simulink model "MotorCC_V3_R2024b"  (R2024b)
settings: Solver=VariableStepAuto  StartTime=0.0  StopTime=inf  RelTol=1e-3
undefined symbols (not defined in the file or in its folder): LF
libraries: instrumentseriallib x3
settings Model: PacingRate=0.010000  Creator=ignacioalvarado  LastModifiedBy=ignacio
settings OptimizationCC: ReuseModelBlockBuffer=off
settings RTWCC: GPUComputeCapability=3.5
settings ConfigComp: CovBoundaryAbsTol=1.0e-5

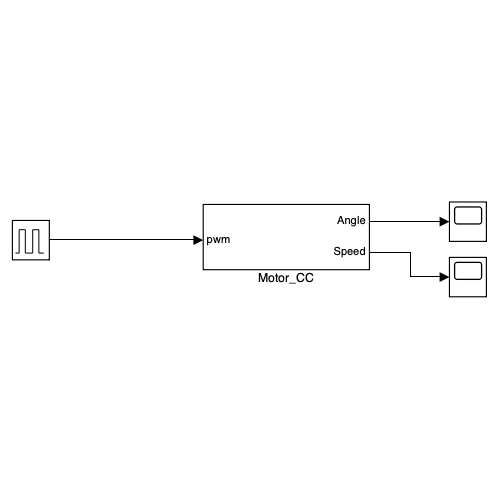
[thumbnail: Simulink's stored preview of the top-level diagram]
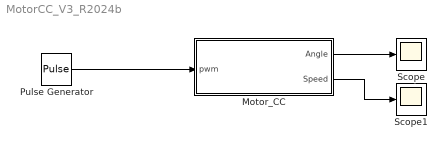
== system MotorCC_V3_R2024b ==
  Motor_CC : Subsystem  InitFcn=|  mask{PortName=Select a serial port}
      | if ismember(get_param(gcb, 'PortName'), {'Select a serial port', 'No serial ports available'})
      |     error('MotorCC:NoSerialPort', 'Connect the Arduino and select its serial port in Motor_CC before running.');
      | end
      mask prompts: PortName "Arduino Port:"
      mask init:
      | % Pass the chosen port to all three Instrument Control Toolbox blocks.
      | block = gcb;
      | selected = get_param(block, 'PortName');
      | if ~ismember(selected, {'Select a serial port', 'No serial ports available'})
      |     set_param([block '/Serial Configuration'], 'Port', selected);
      |     set_param([block '/Serial Send'], 'Port', selected);
      |     set_param([block '/Serial Receive'], 'Port', selected);
      | end
      settings: OpenFcn=|
      | % Refresh the list before showing the mask.
      | block = gcb;
      | if strcmp(get_param(bdroot(block), 'SimulationStatus'), 'stopped')
      |     ports = serialportlist('available');
      |     if isempty(ports)
      |         options = {'No serial ports available'};
      |     else
      |         options = [{'Select a serial port'}, cellstr(ports(:).')];
      |     end
      |     mask = Simulink.Mask.get(block);
      |     port = mask.getParameter('PortName');
      |     selected = get_param(block, 'PortName');
      |     port.TypeOptions = options;
      |     if ~ismember(selected, options)
      |         set_param(block, 'PortName', options{1});
      |     end
      | end
      | open_system(block, 'mask');
      mask TypeOptions PortName: Select a serial port | /dev/tty.Bluetooth-Incoming-Port | /dev/cu.Bluetooth-Incoming-Port | /dev/tty.usbmodem141011 | /dev/cu.usbmodem141011
  Pulse Generator : DiscretePulseGenerator  PulseType=Time based  Amplitude=50  Period=10  PulseWidth=50
  Scope : Scope
  Scope1 : Scope
  wires:
  Pulse Generator/1 -> Motor_CC/1(pwm)
  Motor_CC/1(Angle) -> Scope/1
  Motor_CC/2(Speed) -> Scope1/1

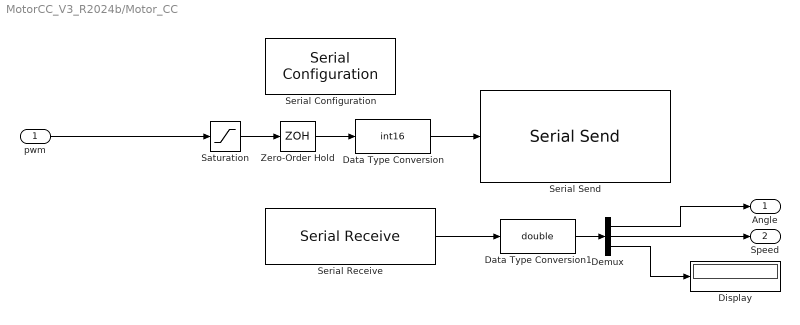
== system MotorCC_V3_R2024b/Motor_CC ==
  pwm : Inport
  Data Type Conversion : DataTypeConversion  OutDataTypeStr=int16  SaturateOnIntegerOverflow=off  RndMeth=Floor  LockScale=on
  Data Type Conversion1 : DataTypeConversion  OutDataTypeStr=double  SaturateOnIntegerOverflow=off  RndMeth=Floor
  Demux : Demux  Outputs=3
  Display : Display
  Saturation : Saturate  UpperLimit=255  LowerLimit=-255
  Serial Configuration : instrumentseriallib/Serial Configuration  Priority=-200000  PortSel=/dev/cu.usbmodem23101  Port=/dev/cu.usbmodem23101  ComPort=/dev/cu.usbmodem23101  BaudRate=115200  DataBits=8  Parity=none  StopBits=1  ByteOrder=little-endian  FlowControl=none  Timeout=10  SimulateUsing=Interpreted execution  BlockInModel=on  aMode=1
  Serial Receive : instrumentseriallib/Serial Receive  Priority=1  PortSel=/dev/cu.usbmodem23101  Port=/dev/cu.usbmodem23101  ComPort=/dev/cu.usbmodem23101  DataType=single  SaveDataType=uint8  ToggleHeader=on  Header='V'  ToggleDataSize=on  DataSize=[1 3]  ToggleTerminator=on  Terminator=LF ('\n')  CustomTerminator=[]  InputFormat=Row major  EnableBlockingMode=on  ActionDataUnavailable=Output last received value  ActionWhenDataUnavailable=Output last received value  CustomValue=0  SampleTime=0.01  SimulateUsing=Interpreted execution  BlockInModel=on  aMode=1
  Serial Send : instrumentseriallib/Serial Send  Priority=1  PortSel=/dev/cu.usbmodem23101  Port=/dev/cu.usbmodem23101  ComPort=/dev/cu.usbmodem23101  Header='A'  Terminator=LF ('\n')  CustomTerminator=[]  EnableBlockingMode=on  SimulateUsing=Interpreted execution  BlockInModel=on  aMode=1
  Zero-Order Hold : ZeroOrderHold  SampleTime=0.01
  Angle : Outport
  Speed : Outport  Port=2
  wires:
  Serial Receive/1 -> Data Type Conversion1/1
  Data Type Conversion/1 -> Serial Send/1
  pwm/1 -> Saturation/1
  Zero-Order Hold/1 -> Data Type Conversion/1
  Saturation/1 -> Zero-Order Hold/1
  Data Type Conversion1/1 -> Demux/1
  Demux/2 -> Speed/1
  Demux/1 -> Angle/1
  Demux/3 -> Display/1
